simulink model "CIFB3_General"  (R2022b)
settings: Solver=FixedStepDiscrete  StartTime=0.0  StopTime=0.01  RelTol=1e-3
libraries: dspsrcs4 x1
settings Model: Creator=ASAA  LastModifiedBy=ASAA

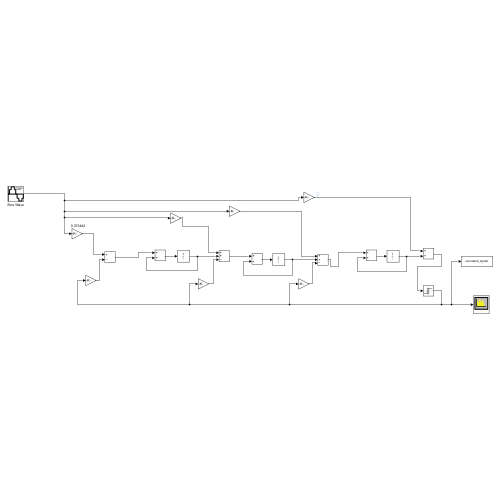
[thumbnail: Simulink's stored preview of the top-level diagram]
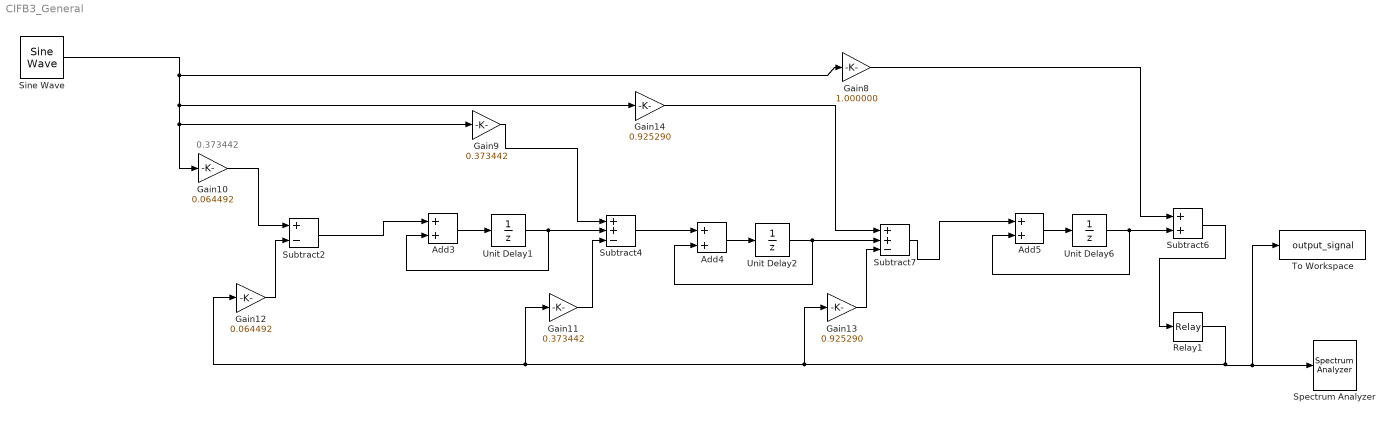
== system CIFB3_General ==
  note: 0.373442
  Add3 : Sum
  Add4 : Sum
  Add5 : Sum
  Gain10 : Gain  Gain=0.064492
  Gain11 : Gain  Gain=0.373442
  Gain12 : Gain  Gain=0.064492
  Gain13 : Gain  Gain=0.925290
  Gain14 : Gain  Gain=0.925290
  Gain8 : Gain  Gain=1.000000
  Gain9 : Gain  Gain=0.373442
  Relay1 : Relay  OffOutputValue=-1
  Sine Wave : dspsrcs4/Sine Wave  Amplitude=0.63  Frequency=100e3  Phase=0  SampleMode=Discrete  OutComplex=Real  CompMethod=Trigonometric fcn  TableSize=Speed  SampleTime=1e-8  SamplesPerFrame=1  ResetState=Restart at time zero  OutputFrames=off  dataType=double  wordLen=16  udDataType=sfix(16)  fracBitsMode=Best precision  numFracBits=15  OutDataTypeStr=double  LastOutDataTypeStr=double
  Spectrum Analyzer : SpectrumAnalyzer
  Subtract2 : Sum  Inputs=+-
  Subtract4 : Sum  Inputs=++-
  Subtract6 : Sum
  Subtract7 : Sum  Inputs=++-
  To Workspace : ToWorkspace  VariableName=output_signal  SaveFormat=Timeseries  SampleTime=-1
  Unit Delay1 : UnitDelay  SampleTime=1/100e6  HasFrameUpgradeWarning=on
  Unit Delay2 : UnitDelay  SampleTime=1/100e6  HasFrameUpgradeWarning=on
  Unit Delay6 : UnitDelay  SampleTime=1/100e6  HasFrameUpgradeWarning=on
  wires:
  Unit Delay6/1 -> Subtract6/2, Add5/2
  Subtract7/1 -> Add5/1
  Add5/1 -> Unit Delay6/1
  Add3/1 -> Unit Delay1/1
  Subtract6/1 -> Relay1/1
  Gain11/1 -> Subtract4/3
  Gain9/1 -> Subtract4/1
  Subtract4/1 -> Add4/1
  Gain12/1 -> Subtract2/2
  Gain10/1 -> Subtract2/1
  Subtract2/1 -> Add3/1
  Relay1/1 -> To Workspace/1, Spectrum Analyzer/1, Gain12/1, Gain11/1, Gain13/1
  Sine Wave/1 -> Gain8/1, Gain14/1, Gain9/1, Gain10/1
  Add4/1 -> Unit Delay2/1
  Gain13/1 -> Subtract7/3
  Gain14/1 -> Subtract7/1
  Unit Delay1/1 -> Subtract4/2, Add3/2
  Unit Delay2/1 -> Subtract7/2, Add4/2
  Gain8/1 -> Subtract6/1
